simulink model "PDW_System_F04"  (R2022b)
settings: Solver=FixedStepDiscrete  StartTime=0.0  StopTime=4.8  FixedStep=0.02  RelTol=1e-3
undefined symbols (not defined in the file or in its folder): DiscIntNeverNeededParam
settings Model: Creator=chaym  LastModifiedBy=chaym

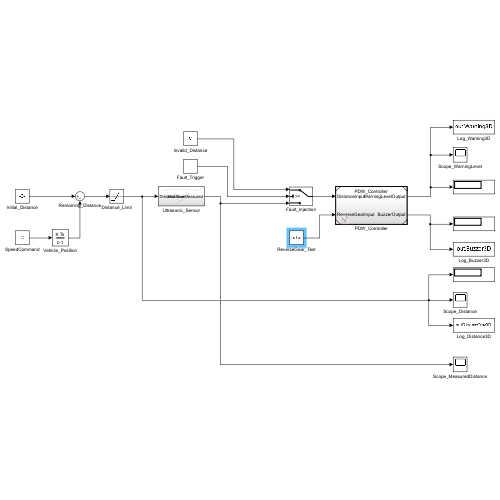
[thumbnail: Simulink's stored preview of the top-level diagram]
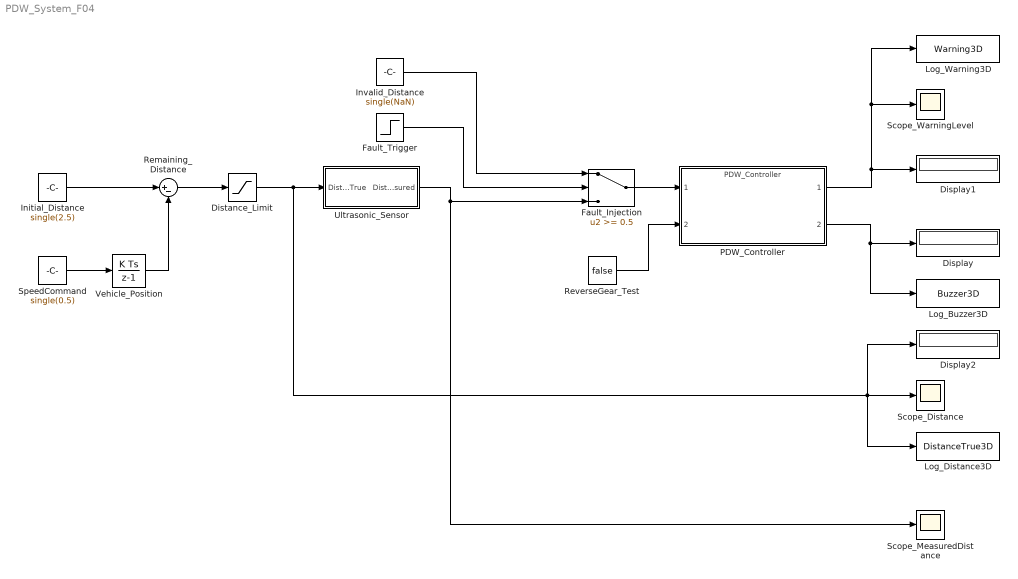
== system PDW_System_F04 ==
  Display : Display
  Display1 : Display
  Display2 : Display
  Distance_Limit : Saturate  UpperLimit=4  LowerLimit=0
  Fault_Injection : Switch  Threshold=0.5  SaturateOnIntegerOverflow=off  InputSameDT=off
  Fault_Trigger : Step  Time=10  SampleTime=0.02
  Initial_Distance : Constant  Value=single(2.5)
  Invalid_Distance : Constant  Value=single(NaN)
  Log_Buzzer3D : ToWorkspace  VariableName=Buzzer3D  SaveFormat=Timeseries  SampleTime=-1
  Log_Distance3D : ToWorkspace  VariableName=DistanceTrue3D  SaveFormat=Timeseries  SampleTime=-1
  Log_Warning3D : ToWorkspace  VariableName=Warning3D  SaveFormat=Timeseries  SampleTime=-1
  PDW_Controller : ModelReference  ModelNameDialog=PDW_Controller  SimulationMode=Normal  ModelReferenceVersion=1.31
  Remaining_Distance : Sum  Inputs=|+-
  ReverseGear_Test : Constant  Value=false  OutDataTypeStr=boolean
  Scope_Distance : Scope
  Scope_MeasuredDistance : Scope
  Scope_WarningLevel : Scope
  SpeedCommand : Constant  Value=single(0.5)
  Ultrasonic_Sensor : Subsystem
  Vehicle_Position : DiscreteIntegrator  SampleTime=0.02  ICPrevOutput=DiscIntNeverNeededParam  ICPrevScaledInput=DiscIntNeverNeededParam
  wires:
  SpeedCommand/1 -> Vehicle_Position/1
  Initial_Distance/1 -> Remaining_Distance/1
  Vehicle_Position/1 -> Remaining_Distance/2
  Remaining_Distance/1 -> Distance_Limit/1
  Distance_Limit/1 -> Ultrasonic_Sensor/1(DistanceTrue), Display2/1, Log_Distance3D/1, Scope_Distance/1
  ReverseGear_Test/1 -> PDW_Controller/2
  PDW_Controller/1 -> Scope_WarningLevel/1, Log_Warning3D/1, Display1/1
  PDW_Controller/2 -> Log_Buzzer3D/1, Display/1
  Ultrasonic_Sensor/1(DistanceMeasured) -> Scope_MeasuredDistance/1, Fault_Injection/3
  Invalid_Distance/1 -> Fault_Injection/1
  Fault_Trigger/1 -> Fault_Injection/2
  Fault_Injection/1 -> PDW_Controller/1

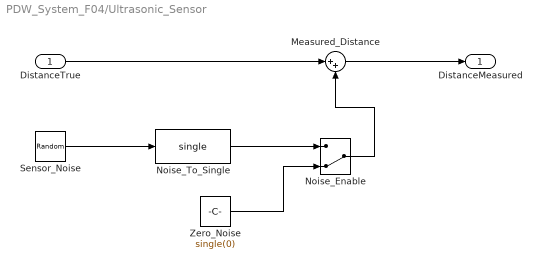
== system PDW_System_F04/Ultrasonic_Sensor ==
  DistanceTrue : Inport
  Measured_Distance : Sum  Inputs=|++
  Noise_Enable : ManualSwitch  CurrentSetting=0
  Noise_To_Single : DataTypeConversion  OutDataTypeStr=single  SaturateOnIntegerOverflow=off  RndMeth=Floor
  Sensor_Noise : RandomNumber  Variance=0.0001  Seed=12345  SampleTime=0.02
  Zero_Noise : Constant  Value=single(0)
  DistanceMeasured : Outport
  wires:
  DistanceTrue/1 -> Measured_Distance/1
  Sensor_Noise/1 -> Noise_To_Single/1
  Noise_To_Single/1 -> Noise_Enable/1
  Zero_Noise/1 -> Noise_Enable/2
  Noise_Enable/1 -> Measured_Distance/2
  Measured_Distance/1 -> DistanceMeasured/1
